simulink model "LQI2_tests"  (R2026a)
settings: Solver=FixedStepAuto  StopTime=35  FixedStep=1e-3  RelTol=1e-5
values from neighbouring files (symbols this model uses):
  A_i = blkdiag(zeros(3), A_iPrime)    [LQIDevR2.m]    (also in LQIDevR3.m = zeros(4); RSDDevR1.m = [ 0 1)
  B_i = [eye(3) ... (first row only)    [LQIDevR2.m]    (also in LQIDevR3.m)
  g = p.g    [HopperLinearization_6DOF.m]    (also in HopperLinearization_6DOF_LQR.m; HopperLinearization_6DOF_inertial.m; HopperLinearization_errorq.m; HopperLinearization_lqi.m = par.g)
  m = p.m    [HopperLinearization_6DOF.m]    (also in HopperLinearization_6DOF_LQR.m = 114; HopperLinearization_6DOF_inertial.m = mass; HopperLinearization_errorq.m = mass; HopperLinearization_lqi.m = mass)
  omega_1 = 2*pi/54    (= 0.116355283466)    [LQIDevR2.m]
  params = struct()    [GenerateLQ.m]    (also in LQGeneral.m; LQIDevR1.m; LQIDevR2.m; LQIDevR3.m)
undefined symbols (not defined in the file or in its folder): IN, Klqi, VEH
libraries: simulink_extras x3, aerolibanim x1, matrix_library x1
settings Model: Creator=asing  LastModifiedBy=maxma
settings DebuggingCC: SignalInfNanChecking=warning
settings SimscapeCC: SimscapeNominalValues="[{\"value\":\"1\",\"unit\":\"A\"},{\"value\":\"1\",\"unit\":\"bar\"},{\"value\":\"1\",\"unit\":\"cm^2\"},{\"value\":\"1\",\"unit\":\"cm^3/s\"},{\"value\":\"1\",\"unit\":\"kJ/kg\"},{\"value\":\"1\",\"unit\":\"kW\"},{\"value\":\"1\",\"unit\":\"l\"},{\"value\":\"1\",\"unit\":\"N\"},{\"value\":\"1\",\"unit\":\"N*m\"},{\"value\":\"1\",\"unit\":\"V\"}]"  SimscapeLogType=none  SimscapeLogDataHistory=5000.0

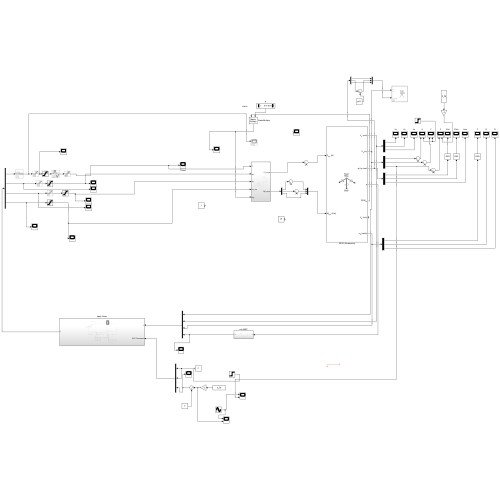
[thumbnail: Simulink's stored preview of the top-level diagram]
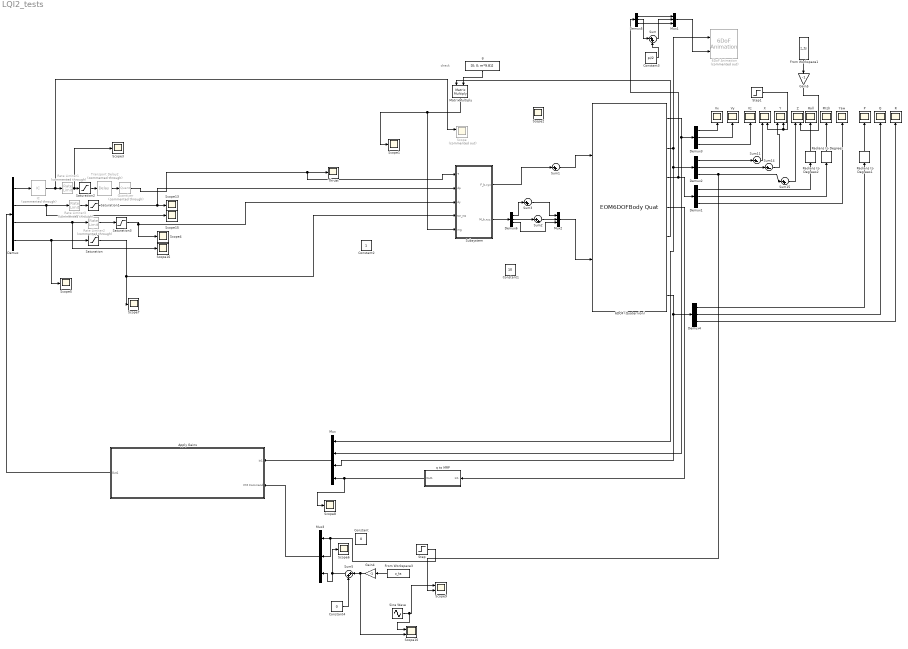
== system LQI2_tests ==
  note: check
  6DOF (Quaternion) : EOM6DOFBodyQuat  mass_0=m  inertia=params.I
  6DoF Animation : aerolibanim/6DoF Animation  Commented=on  u1=[0 200 -200 200 -100 5]  u2=0.1  u3=2  u4=[4000 0 -5000]  u5=Fixed position  u6=[100 100 -50]  u7=10  u8=on
  Apply Gains : Subsystem
  Constant : Constant  Value=0
  Constant1 : Constant  Value=10
  Constant2 : Constant
  Constant3 : Constant  Value=pi/2
  Constant4 : Constant  Value=0
  Demux : Demux
  Demux{1..6} (6 alike) : Demux  Outputs=3
  From Workspace1 : FromWorkspace  VariableName=z_ts
  From Workspace3 : FromWorkspace  VariableName=z_ts
  Gain4 : Gain  Gain=-1
  Gain5 : Gain  Gain=-1
  IC : InitialCondition  Commented=through  Value=VEH.mass.wet*g
  MatrixMultiply : Product  Multiplication=Matrix(*)
  Mux : Mux
  Mux1 : Mux  Inputs=3
  Mux2 : Mux  Inputs=3
  Mux3 : Mux  Inputs=3
  P : Scope
      settings: ActiveDisplayYMinimum=-13827.727177361454  ActiveDisplayYMaximum=124449.54459625312  DataLoggingVariableName=ScopeData9
  Pitch : Scope
      settings: ActiveDisplayYMinimum=-4.900529428260505  ActiveDisplayYMaximum=4.3505112101193859  DataLoggingVariableName=ScopeData4
  Q : Scope
      settings: ActiveDisplayYMinimum=-42.430641246985132  ActiveDisplayYMaximum=42.428715698043774  DataLoggingVariableName=ScopeData10
  Quantizer : Quantizer  Commented=through  QuantizationInterval=IN.throttle_valve.resolution
  R : Scope
      settings: ActiveDisplayYMinimum=-0.0070860969112896514  ActiveDisplayYMaximum=0.0085398632976064828  DataLoggingVariableName=ScopeData11
  Radians to Degrees : simulink_extras/Transformations/Radians to Degrees
  Radians to Degrees1 : simulink_extras/Transformations/Radians to Degrees
  Radians to Degrees2 : simulink_extras/Transformations/Radians to Degrees
  Rate Limiter1 : RateLimiter  Commented=through  RisingSlewLimit=10  FallingSlewLimit=-10  SampleTimeMode=inherited
  Rate Limiter2 : RateLimiter  Commented=through  RisingSlewLimit=pi/16  FallingSlewLimit=-pi/16  SampleTimeMode=inherited
  Rate Limiter3 : RateLimiter  Commented=through  RisingSlewLimit=pi/16  FallingSlewLimit=-pi/16  SampleTimeMode=inherited
  Roll : Scope
      settings: ActiveDisplayYMinimum=-4.4001681125980641  ActiveDisplayYMaximum=5.4626026187327055  DataLoggingVariableName=ScopeData3
  Saturation : Saturate  UpperLimit=50  LowerLimit=-50
  Saturation1 : Saturate  UpperLimit=pi/16  LowerLimit=-pi/16
  Saturation2 : Saturate  UpperLimit=2600  LowerLimit=800
  Saturation3 : Saturate  UpperLimit=pi/16  LowerLimit=-pi/16
  Scope : Scope  Commented=on  NumInputPorts=2
      settings: ActiveDisplayYMinimum=725.64918679567745  ActiveDisplayYMaximum=1423.3753088923004  DataLoggingVariableName=ScopeData52
  Scope{1..8,13,15..16} (11 alike) : Scope
      Scope1 settings: ActiveDisplayYMinimum=-1  ActiveDisplayYMaximum=1  DataLoggingVariableName=ScopeData31
      Scope13 settings: ActiveDisplayYMinimum=-0.0014103158373404341  ActiveDisplayYMaximum=0.0013269104944431994  DataLoggingVariableName=ScopeData32
      Scope15 settings: ActiveDisplayYMinimum=-0.0031488454332496813  ActiveDisplayYMaximum=0.0026869300038082061  DataLoggingVariableName=ScopeData33
      Scope16 settings: ActiveDisplayYMinimum=-0.002689460767411929  ActiveDisplayYMaximum=0.0031507068883406507  DataLoggingVariableName=ScopeData34
      Scope2 settings: ActiveDisplayYMinimum=-1  ActiveDisplayYMaximum=1  DataLoggingVariableName=ScopeData16
      Scope3 settings: ActiveDisplayYMinimum=-3.0138014269044207E-7  ActiveDisplayYMaximum=2.7124212842139794E-6  DataLoggingVariableName=ScopeData17
      Scope4 settings: ActiveDisplayYMinimum=-0.0013277363090328841  ActiveDisplayYMaximum=0.0014109778865573151  DataLoggingVariableName=ScopeData18
      Scope5 settings: ActiveDisplayYMinimum=-59.073001162491146  ActiveDisplayYMaximum=98.278860989440048  DataLoggingVariableName=ScopeData27
      Scope6 settings: ActiveDisplayYMinimum=-58.523257369563716  ActiveDisplayYMaximum=6.7093163260734654  DataLoggingVariableName=ScopeData12
      Scope7 settings: ActiveDisplayYMinimum=-1.3476077084435787E-16  ActiveDisplayYMaximum=1.0641031604675325E-16  DataLoggingVariableName=ScopeData62
      Scope8 settings: ActiveDisplayYMinimum=-0.023240810681171287  ActiveDisplayYMaximum=0.015298204339471872  DataLoggingVariableName=ScopeData92
  Scope10 : Scope  NumInputPorts=2
      settings: ActiveDisplayYMinimum=-1  ActiveDisplayYMaximum=1  DataLoggingVariableName=ScopeData15
  Scope9 : Scope  NumInputPorts=2
      settings: ActiveDisplayYMinimum=-64.791663560954277  ActiveDisplayYMaximum=62.754629284550475  DataLoggingVariableName=ScopeData13
  Sine Wave : Sin  Amplitude=-50  Frequency=(2*pi)/45  SampleTime=0
  Step : Step  Time=10  FinalValue=10  SampleTime=0
  Step1 : Step  Time=10  FinalValue=3  SampleTime=0
  Subsystem : Subsystem
  Sum{,1..3,5,15} (6 alike) : Sum  Inputs=|++
  Sum11 : Sum  Inputs=|+-
  Sum14 : Sum  Inputs=|+-
  Thrust : Scope
      settings: ActiveDisplayYMinimum=575  ActiveDisplayYMaximum=2825  DataLoggingVariableName=ScopeData25
  Transport Delay2 : TransportDelay  Commented=through  DelayTime=IN.throttle_valve_latency
  Vx : Scope
      settings: ActiveDisplayYMinimum=-63.872379284445891  ActiveDisplayYMaximum=574.47074934538614  DataLoggingVariableName=ScopeData6
  Vy : Scope
      settings: ActiveDisplayYMinimum=-1  ActiveDisplayYMaximum=1  DataLoggingVariableName=ScopeData7
  Vz : Scope
      settings: ActiveDisplayYMinimum=-10.20538653153435  ActiveDisplayYMaximum=9.6433449078999853  DataLoggingVariableName=ScopeData8
  X : Scope  NumInputPorts=2
      settings: ActiveDisplayYMinimum=-1.4064408221254825  ActiveDisplayYMaximum=12.652876209185806
  Y : Scope  NumInputPorts=2
      settings: ActiveDisplayYMinimum=-1.4062487407024427  ActiveDisplayYMaximum=12.651159585426942
  Yaw : Scope
      settings: ActiveDisplayYMinimum=-0.00340579602696374  ActiveDisplayYMaximum=0.0019397588185685647  DataLoggingVariableName=ScopeData5
  Z : Scope  NumInputPorts=2
      settings: ActiveDisplayYMinimum=-58.57222786375106  ActiveDisplayYMaximum=6.77488522137757  DataLoggingVariableName=ScopeData2
  g : Constant  Value=[0; 0; m*9.81]
  q to MRP : Subsystem
  wires:
  6DOF (Quaternion)/3 -> Demux5/1, Demux1/1
  Demux1/2 -> Radians to Degrees/1
  Demux3/1 -> Vx/1
  Demux3/2 -> Vy/1
  Demux4/1 -> Radians to Degrees1/1
  Demux4/2 -> Q/1
  Demux4/3 -> R/1
  Demux3/3 -> Vz/1
  Demux1/1 -> Radians to Degrees2/1
  Demux1/3 -> Yaw/1
  g/1 -> MatrixMultiply/2
  Rate Limiter1/1 -> Scope3/1, Saturation2/1
  Demux/2 -> Rate Limiter3/1, Scope15/1
  Demux/1 -> IC/1
  Transport Delay2/1 -> Quantizer/1
  IC/1 -> Scope/1, Rate Limiter1/1
  6DOF (Quaternion)/1 -> Mux/2, Demux3/1
  6DOF (Quaternion)/2 -> Mux/1, Demux2/1, 6DoF Animation/1
  Saturation2/1 -> Transport Delay2/1
  Demux2/1 -> Sum11/1
  Demux2/2 -> Sum14/1
  Sum14/1 -> Y/1
  Demux2/3 -> Scope9/2, Sum15/1
  Demux/4 -> Scope5/1, Saturation/1
  Radians to Degrees/1 -> Pitch/1
  Sum15/1 -> Z/1
  Radians to Degrees1/1 -> P/1
  Radians to Degrees2/1 -> Roll/1
  6DOF (Quaternion)/5 -> MatrixMultiply/1
  Quantizer/1 -> Subsystem/1(T), Thrust/1
  Demux/3 -> Scope16/1, Rate Limiter2/1
  Apply Gains/1(Out1) -> Demux/1
  Sum11/1 -> X/1
  MatrixMultiply/1 -> Subsystem/5(mg), Scope1/1
  Saturation/1 -> Subsystem/4(tor_rcs), Scope7/1
  Saturation3/1 -> Subsystem/3(dy), Scope4/1
  6DOF (Quaternion)/7 -> Mux/3, Demux4/1
  Saturation1/1 -> Subsystem/2(dp), Scope13/1
  Rate Limiter3/1 -> Saturation1/1
  Rate Limiter2/1 -> Saturation3/1
  From Workspace3/1 -> Gain4/1
  Mux3/1 -> Apply Gains/2(XYZ Command)
  Mux/1 -> Apply Gains/1(In1)
  q to MRP/1(Out1) -> Scope8/1, Mux/4
  From Workspace1/1 -> Gain5/1
  6DOF (Quaternion)/4 -> q to MRP/1(In1)
  Constant3/1 -> Sum/2
  Sum/1 -> Mux1/2
  Demux5/2 -> Sum/1
  Demux5/1 -> Mux1/1
  Demux5/3 -> Mux1/3
  Mux1/1 -> 6DoF Animation/2
  Step1/1 -> Y/2, X/2
  Subsystem/1(F_b,xyz) -> Sum1/1
  Sum1/1 -> 6DOF (Quaternion)/1
  Subsystem/2(M_b,xyz) -> Demux6/1
  Demux6/2 -> Sum2/1
  Sum2/1 -> Mux2/2
  Mux2/1 -> 6DOF (Quaternion)/2
  Sum3/1 -> Mux2/1
  Demux6/1 -> Sum3/1
  Demux6/3 -> Mux2/3
  Gain4/1 -> Scope10/2, Sum5/1
  Constant4/1 -> Sum5/2
  Sum5/1 -> Mux3/3, Scope6/1
  Step/1 -> Mux3/2, Mux3/1
  Sine Wave/1 -> Scope10/1, Scope9/1
  ? -> ?
  Gain5/1 -> Z/2

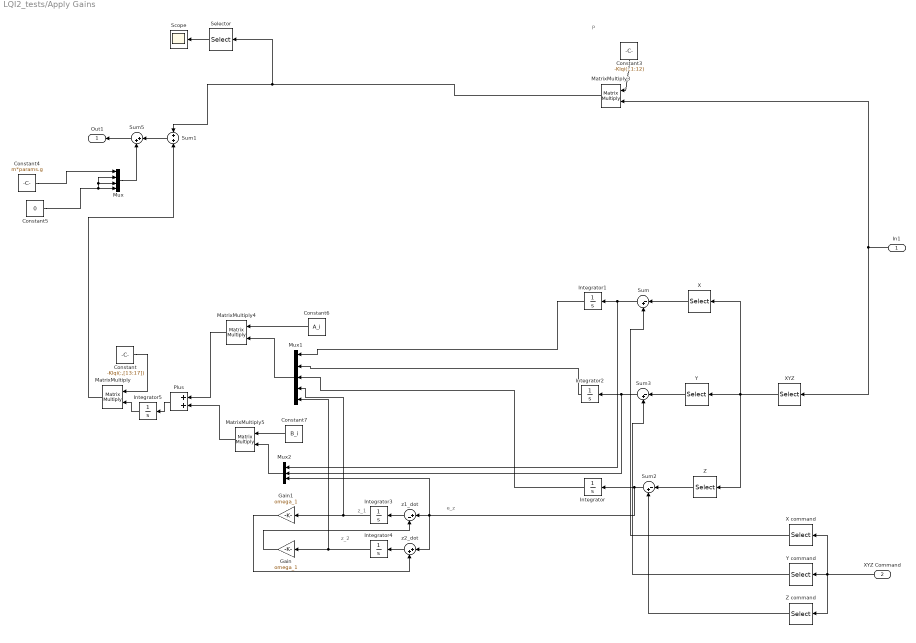
== system LQI2_tests/Apply Gains ==
  note: e_z
  note: z_1
  note: P
  note: z_2
  In1 : Inport
  XYZ Command : Inport  Port=2
  Constant : Constant  Value=-Klqi(:,[13:17])
  Constant3 : Constant  Value=-Klqi(:,1:12)
  Constant4 : Constant  Value=m*params.g
  Constant5 : Constant  Value=0
  Constant6 : Constant  Value=A_i
  Constant7 : Constant  Value=B_i
  Gain : Gain  Gain=omega_1
  Gain1 : Gain  Gain=omega_1
  Integrator{,1..5} (6 alike) : Integrator
  MatrixMultiply{,3..5} (4 alike) : Product  Multiplication=Matrix(*)
  Mux : Mux
  Mux1 : Mux  Inputs=5
  Mux2 : Mux  Inputs=3
  Plus : Sum
  Scope : Scope
      settings: ActiveDisplayYMinimum=-1.4616719400156864E-13  ActiveDisplayYMaximum=1.7248708805376873E-13  DataLoggingVariableName=ScopeData19
  Selector : Selector  InputPortWidth=4  IndexOptions=Index vector (dialog)  Indices=[2 3]  OutputSizes=1
  Sum : Sum  Inputs=|-+
  Sum1 : Sum  Inputs=+|+
  Sum2 : Sum  Inputs=|-+
  Sum3 : Sum  Inputs=|-+
  Sum5 : Sum  Inputs=|++
  X : Selector  InputPortWidth=3  IndexOptions=Index vector (dialog)  Indices=[1 ]  OutputSizes=1
  X command : Selector  InputPortWidth=3  IndexOptions=Index vector (dialog)  Indices=[1 ]  OutputSizes=1
  XYZ : Selector  InputPortWidth=12  IndexOptions=Index vector (dialog)  Indices=[1 2 3]  OutputSizes=1
  Y : Selector  InputPortWidth=3  IndexOptions=Index vector (dialog)  Indices=[2 ]  OutputSizes=1
  Y command : Selector  InputPortWidth=3  IndexOptions=Index vector (dialog)  Indices=[2 ]  OutputSizes=1
  Z : Selector  InputPortWidth=3  IndexOptions=Index vector (dialog)  Indices=[3 ]  OutputSizes=1
  Z command : Selector  InputPortWidth=3  IndexOptions=Index vector (dialog)  Indices=[3 ]  OutputSizes=1
  z1_dot : Sum  Inputs=|+-
  z2_dot : Sum  Inputs=|++
  Out1 : Outport
  wires:
  Integrator/1 -> Mux1/3
  Integrator2/1 -> Mux1/2
  Integrator1/1 -> Mux1/1
  XYZ/1 -> Z/1, X/1, Y/1
  Constant3/1 -> MatrixMultiply3/1
  In1/1 -> XYZ/1, MatrixMultiply3/2
  Sum/1 -> Mux2/1, Integrator1/1
  Z/1 -> Sum2/1
  Sum2/1 -> Mux2/3, z2_dot/1, z1_dot/1, Integrator/1
  X/1 -> Sum/1
  Y/1 -> Sum3/1
  Sum3/1 -> Mux2/2, Integrator2/1
  XYZ Command/1 -> Z command/1, X command/1, Y command/1
  X command/1 -> Sum/2
  Y command/1 -> Sum3/2
  Z command/1 -> Sum2/2
  MatrixMultiply3/1 -> Sum1/1, Selector/1
  Selector/1 -> Scope/1
  Sum1/1 -> Sum5/1
  Sum5/1 -> Out1/1
  Mux/1 -> Sum5/2
  Constant5/1 -> Mux/2, Mux/3, Mux/4
  Constant4/1 -> Mux/1
  Constant6/1 -> MatrixMultiply4/1
  Constant7/1 -> MatrixMultiply5/1
  MatrixMultiply4/1 -> Plus/1
  MatrixMultiply5/1 -> Plus/2
  z1_dot/1 -> Integrator3/1
  z2_dot/1 -> Integrator4/1
  Integrator4/1 -> Gain/1, Mux1/5
  Integrator3/1 -> Gain1/1, Mux1/4
  Gain/1 -> z1_dot/2
  Gain1/1 -> z2_dot/2
  Mux1/1 -> MatrixMultiply4/2
  Mux2/1 -> MatrixMultiply5/2
  Constant/1 -> MatrixMultiply/1
  MatrixMultiply/1 -> Sum1/2
  Plus/1 -> Integrator5/1
  Integrator5/1 -> MatrixMultiply/2

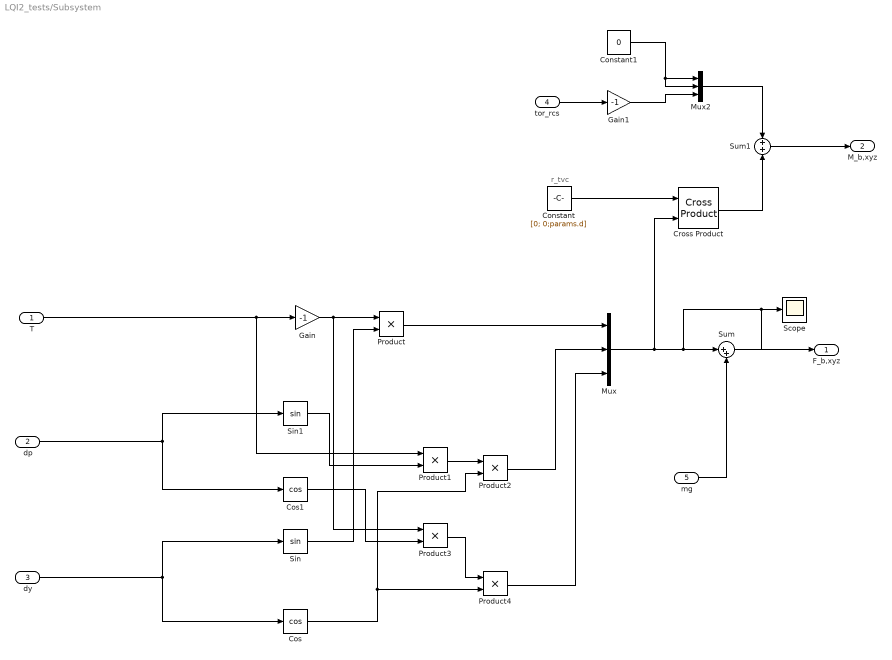
== system LQI2_tests/Subsystem ==
  note: r_tvc
  T : Inport
  dp : Inport  Port=2
  dy : Inport  Port=3
  tor_rcs : Inport  Port=4
  mg : Inport  Port=5
  Constant : Constant  Value=[0; 0;params.d]
  Constant1 : Constant  Value=0
  Cos : Trigonometry  Operator=cos
  Cos1 : Trigonometry  Operator=cos
  Cross Product : matrix_library/Cross Product
  Gain : Gain  Gain=-1
  Gain1 : Gain  Gain=-1
  Mux : Mux  Inputs=3
  Mux2 : Mux  Inputs=3
  Product{,1..4} (5 alike) : Product
  Scope : Scope
      settings: ActiveDisplayYMinimum=-1457.8565194744922  ActiveDisplayYMaximum=161.02888108059477  DataLoggingVariableName=ScopeData14
  Sin : Trigonometry
  Sin1 : Trigonometry
  Sum : Sum  Inputs=|++
  Sum1 : Sum  Inputs=+|+
  F_b,xyz : Outport
  M_b,xyz : Outport  Port=2
  wires:
  T/1 -> Product1/1, Gain/1
  dy/1 -> Cos/1, Sin/1
  Gain/1 -> Product3/1, Product/1
  Sin/1 -> Product/2
  Product/1 -> Mux/1
  dp/1 -> Cos1/1, Sin1/1
  Sin1/1 -> Product1/2
  Cos/1 -> Product4/2, Product2/2
  Product1/1 -> Product2/1
  Cos1/1 -> Product3/2
  Product3/1 -> Product4/1
  Product4/1 -> Mux/3
  Product2/1 -> Mux/2
  Mux/1 -> Scope/1, Sum/1, Cross Product/2
  Constant/1 -> Cross Product/1
  mg/1 -> Sum/2
  Constant1/1 -> Mux2/2, Mux2/1
  tor_rcs/1 -> Gain1/1
  Mux2/1 -> Sum1/1
  Cross Product/1 -> Sum1/2
  Sum/1 -> F_b,xyz/1
  Sum1/1 -> M_b,xyz/1
  Gain1/1 -> Mux2/3

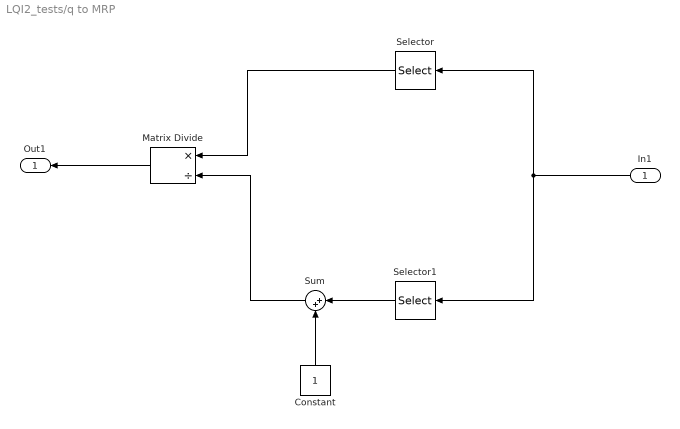
== system LQI2_tests/q to MRP ==
  In1 : Inport
  Constant : Constant
  Matrix Divide : Product  Inputs=*/
  Selector : Selector  InputPortWidth=4  IndexOptions=Index vector (dialog)  Indices=[2 3 4]  OutputSizes=1
  Selector1 : Selector  InputPortWidth=4  IndexOptions=Index vector (dialog)  Indices=[1]  OutputSizes=1
  Sum : Sum  Inputs=|++
  Out1 : Outport
  wires:
  In1/1 -> Selector1/1, Selector/1
  Selector1/1 -> Sum/1
  Constant/1 -> Sum/2
  Selector/1 -> Matrix Divide/1
  Sum/1 -> Matrix Divide/2
  Matrix Divide/1 -> Out1/1
